simulink model "system_model"  (R2025b)
settings: Solver=VariableStepAuto  StartTime=0.0  StopTime=5  RelTol=1e-3
PreLoadFcn:
  | sideswipe_preload
  | sideswipe_config
InitFcn:
  | sideswipe_plant
values from neighbouring files (symbols this model uses):
  A1p = A1    [sideswipe_control.m]
  A2 = [0   1 ... (first row only)    [sideswipe_plant.m]
  a_v = Ts/(tau_v + Ts)    [sideswipe_control.m]
  accel_bias = 0    [sideswipe_control.m]
  accel_noise = 0    [sideswipe_control.m]
  alpha_comp = tau_cf/(tau_cf + Ts)    [sideswipe_control.m]
  B1p = [B1 Bd]    [sideswipe_control.m]
  B2 = [0    0 ... (first row only)    [sideswipe_plant.m]
  C1 = eye(4)    [sideswipe_plant.m]
  C2 = eye(2)    [sideswipe_plant.m]
  cotroller = 1    [sideswipe_control.m]
  D2 = zeros(2)    [sideswipe_plant.m]
  est_mode = 2    [sideswipe_control.m]
  g = 9.81    [sideswipe_params.m]
  gyro_bias = 0    [sideswipe_control.m]
  gyro_drift = 0    [sideswipe_control.m]
  gyro_noise = 0    [sideswipe_control.m]
  h = 0.130    (= 0.13)    [sideswipe_params.m]
  K_lqr = dlqr(s4d.A, s4d.B, QQ, RR)    [sideswipe_control.m]
  K_PWM = 42.5    [sideswipe_params.m]
  Kd_phi = 0.67    [sideswipe_control.m]
  Kd_psi_c = 8    [sideswipe_control.m]
  Kd_x = 0.02    [sideswipe_control.m]
  Ki_psi_c = 0    [sideswipe_control.m]
  Ki_x = 0.005    [sideswipe_control.m]
  Kp_phi = 21    [sideswipe_control.m]
  Kp_psi_c = 80    [sideswipe_control.m]
  Kp_x = 0.02    [sideswipe_control.m]
  n_delay = 0    [sideswipe_control.m]
  phi_dot_ref = 0    [sideswipe_control.m]
  Psi0 = deg2rad(5)    [sideswipe_params.m]
  psi_ref_max = deg2rad(10)    [sideswipe_control.m]
  R = 0.0325    [sideswipe_params.m]
  theta_dot_ref = 0    [sideswipe_control.m]
  Ts = 0.004    [sideswipe_params.m]
  V_dz = 0    [sideswipe_params.m]
  V_sat = 6    [sideswipe_control.m]
  W = 0.068    [sideswipe_params.m]
undefined symbols (not defined in the file or in its folder): DiscIntNeverNeededParam
libraries: simulink x7, simulink_extras x2, slpidlib x1
settings Model: Creator=shukv  LastModifiedBy=shukv

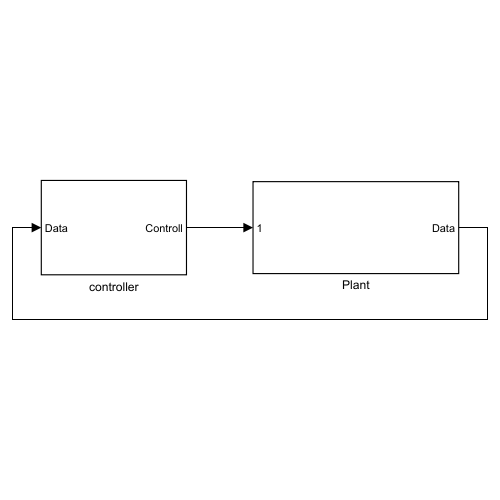
[thumbnail: Simulink's stored preview of the top-level diagram]
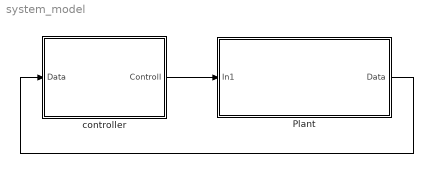
== system system_model ==
  Plant : Subsystem
  controller : Subsystem
  wires:
  controller/1(Controll) -> Plant/1(In1)
  Plant/1(Data) -> controller/1(Data)

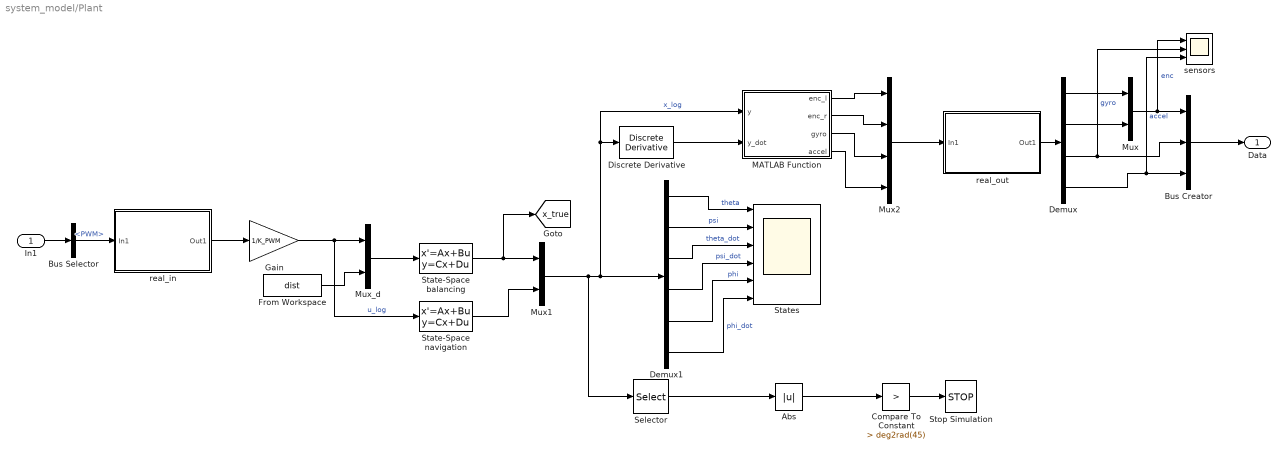
== system system_model/Plant ==
  In1 : Inport
  Abs : Abs  SaturateOnIntegerOverflow=off
  Bus Creator : BusCreator  Inputs=3  OutDataTypeStr=Bus: Data
  Bus Selector : BusSelector  OutputSignals=PWM
  Compare To Constant : simulink/Logic and Bit Operations/Compare To Constant  relop=>  const=deg2rad(45)  OutDataTypeStr=boolean
  Demux : Demux
  Demux1 : Demux  Outputs=6
  Discrete Derivative : simulink/Discrete/Discrete Derivative  gainval=1.0  ICPrevScaledInput=0.0  OutMin=[]  OutMax=[]  OutDataType=fixdt(1, 16)  OutScaling=2^-10  DoSatur=off
  From Workspace : FromWorkspace  VariableName=dist  SampleTime=Ts  Interpolate=off  OutputAfterFinalValue=Holding final value
  Gain : Gain  Gain=1/K_PWM
  MATLAB Function : MATLAB Function  TreatAsAtomicUnit=on
  Mux : Mux  Inputs=2
  Mux1 : Mux  Inputs=2
  Mux2 : Mux
  Mux_d : Mux  Inputs=2
  Selector : Selector  InputPortWidth=6  IndexOptions=Index vector (dialog)  Indices=2  OutputSizes=1
  State-Space balancing : StateSpace  A=A1p  B=B1p  C=C1  D=zeros(4,4)  InitialCondition=[0 Psi0 0 0]
  State-Space navigation : StateSpace  A=A2  B=B2  C=C2  D=D2  InitialCondition=0
  States : Scope  NumInputPorts=6
      settings: ActiveDisplayYMinimum=-1  ActiveDisplayYMaximum=1
  Stop Simulation : Stop
  real_in : Subsystem  Variant=on  EmptyChoice=on
  real_out : Subsystem  Variant=on  EmptyChoice=on
  sensors : Scope  NumInputPorts=3
      settings: ActiveDisplayYMinimum=-1  ActiveDisplayYMaximum=1
  Data : Outport
  tag scope: x_true=global
  wires:
  State-Space navigation/1 -> Mux1/2
  State-Space balancing/1 -> [x_true], Mux1/1
  In1/1 -> Bus Selector/1
  real_in/1(Out1) -> Gain/1
  Bus Selector/1 -> real_in/1(In1)  "<PWM>"
  MATLAB Function/1(enc_l) -> Mux2/1
  From Workspace/1 -> Mux_d/2
  Gain/1 -> State-Space navigation/1, Mux_d/1  "u_log"
  Mux_d/1 -> State-Space balancing/1
  Mux/1 -> sensors/1, Bus Creator/1  "enc"
  Mux1/1 -> Discrete Derivative/1, MATLAB Function/1(y), Demux1/1, Selector/1  "x_log"
  Discrete Derivative/1 -> MATLAB Function/2(y_dot)
  Demux/2 -> Mux/2
  Demux1/5 -> States/5  "phi"
  Demux1/1 -> States/1  "theta"
  Demux/3 -> sensors/2, Bus Creator/2  "gyro"
  Demux1/6 -> States/6  "phi_dot"
  Demux1/2 -> States/2  "psi"
  Demux1/3 -> States/3  "theta_dot"
  Demux1/4 -> States/4  "psi_dot"
  Selector/1 -> Abs/1
  MATLAB Function/2(enc_r) -> Mux2/2
  MATLAB Function/3(gyro) -> Mux2/3
  MATLAB Function/4(accel) -> Mux2/4
  Abs/1 -> Compare To Constant/1
  Mux2/1 -> real_out/1(In1)
  Bus Creator/1 -> Data/1
  Compare To Constant/1 -> Stop Simulation/1
  real_out/1(Out1) -> Demux/1
  Demux/1 -> Mux/1
  Demux/4 -> sensors/3, Bus Creator/3  "accel"

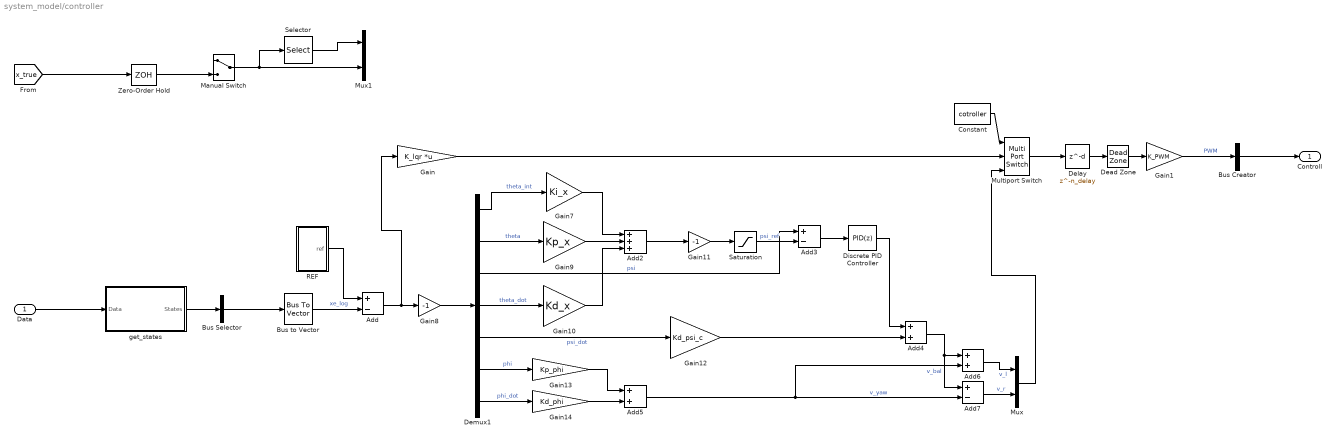
== system system_model/controller ==
  Data : Inport
  Add : Sum  Inputs=+-
  Add2 : Sum  Inputs=+++
  Add3 : Sum  Inputs=+-
  Add4 : Sum
  Add5 : Sum
  Add6 : Sum
  Add7 : Sum  Inputs=+-
  Bus Creator : BusCreator  Inputs=1  OutDataTypeStr=Bus: Controll
  Bus Selector : BusSelector  OutputSignals=theta_int,theta,psi,theta_dot,psi_dot,Phi,phi_dot  OutputAsBus=on
  Bus to Vector : BusToVector
  Constant : Constant  Value=cotroller
  Dead Zone : DeadZone  LowerValue=-V_dz  UpperValue=V_dz
  Delay : Delay  DelayLength=n_delay  SampleTime=Ts
  Demux1 : Demux  Outputs=7
  Discrete PID Controller : slpidlib/PID Controller  Controller=PID  Form=Parallel  TimeDomain=Discrete-time  UseExternalTs=off  SampleTime=Ts  IntegratorMethod=Forward Euler  FilterMethod=Forward Euler  ControllerParametersSource=internal  P=Kp_psi_c  I=Ki_psi_c  UseKiTs=off  D=0  UseExternalDerivativeSource=off  N=100  UseFilter=on  TunerSelectOption=Transfer Function Based (PID Tuner App)  InitialConditionSource=internal  InitialConditionForIntegrator=0  InitialConditionForFilter=0  DifferentiatorICPrevScaledInput=0  ExternalReset=none  TrackingMode=off  Kt=1  LimitOutput=off  SatLimitsSource=internal  UpperSaturationLimit=V_sat  LowerSaturationLimit=-V_sat  LinearizeAsGain=off  AntiWindupMode=clamping  Kb=1  LimitIntegrator=off  UpperIntegratorSaturationLimit=inf  LowerIntegratorSaturationLimit=-inf  POutMin=[]  POutMax=[]  IOutMin=[]  IOutMax=[]  DOutMin=[]  DOutMax=[]  NOutMin=[]  NOutMax=[]  SumOutMin=[]  SumOutMax=[]  SaturationOutMin=[]  SaturationOutMax=[]  PParamMin=[]  PParamMax=[]  IParamMin=[]  IParamMax=[]  DParamMin=[]  DParamMax=[]  NParamMin=[]  NParamMax=[]  KbParamMin=[]  KbParamMax=[]  KtParamMin=[]  KtParamMax=[]  KbOutMin=[]  KbOutMax=[]  KtOutMin=[]  KtOutMax=[]  IntegratorOutMin=[]  IntegratorOutMax=[]  FilterOutMin=[]  FilterOutMax=[]  SumI1OutMin=[]  SumI1OutMax=[]  SumI2OutMin=[]  SumI2OutMax=[]  SumI3OutMin=[]  SumI3OutMax=[]  SumI4OutMin=[]  SumI4OutMax=[]  SumDOutMin=[]  SumDOutMax=[]  DifferentiatorOutMin=[]  DifferentiatorOutMax=[]  FilterDiffOutCoefMin=[]  FilterDiffOutCoefMax=[]  ReciprocalOutMin=[]  ReciprocalOutMax=[]  SumDenOutMin=[]  SumDenOutMax=[]  SumNumOutMin=[]  SumNumOutMax=[]  DivideOutMin=[]  DivideOutMax=[]  UdiffTsProdOutMin=[]  UdiffTsProdOutMax=[]  NTsProdOutMin=[]  NTsProdOutMax=[]  UintegralTsProdOutMin=[]  UintegralTsProdOutMax=[]  UngainTsProdOutMin=[]  UngainTsProdOutMax=[]  ClampingZeroOutDataTypeStr=Inherit: Inherit via back propagation  ClampingZeroOutMin=[]  ClampingZeroOutMax=[]  FilterDenConstantOutDataTypeStr=Inherit: Inherit via back propagation  FilterDenConstantOutMin=[]  FilterDenConstantOutMax=[]  PCopyOutDataTypeStr=Inherit: Inherit via back propagation  PCopyOutMin=[]  PCopyOutMax=[]  NCopyOutDataTypeStr=Inherit: Inherit via back propagation  NCopyOutMin=[]  NCopyOutMax=[]  IntegratorContinuousStateAttributes=''  IntegratorStateMustResolveToSignalObject=off  IntegratorRTWStateStorageClass=Auto  FilterContinuousStateAttributes=''  FilterStateMustResolveToSignalObject=off  FilterRTWStateStorageClass=Auto  ParallelPVariant=InternalParameters  IdealPVariant=Disabled  IVariant=InternalParameters  DVariant=InternalParameters  IntegratorVariant=Discrete  SatVariant=Disabled  AWVariant=Passthrough  PCopyVariant=Disabled  TRVariant=Disabled  FdbkBlocksVariant=Forward  IdealPFdbkVariant=Disabled  SatFdbkVariant=Disabled  DerivativeFilterVariant=ForwardEulerFilter  NVariant=InternalParameters  NCopyVariant=Disabled  FilterICVariant=InternalICsFilter  IntegratorICVariant=InternalICs  ExternalResetVariant=Disabled  TRSumVariant=Passthrough  SumFdbkVariant=Disabled  SumVariant=Sum_PID  TsampFilterVariant=InternalTs  TsampNgainVariant=Passthrough  TsampIntegralVariant=Disabled_SignalSpec  ExternalSaturationOutDataTypeStr=Inherit: Same as second input  DerivativeSourceVariant=ErrorSignal  PreIntVariant=InternalPreInt
      settings: LibrarySourceBlock=simulink/Discrete/Discrete PID Controller
  Gain : Gain  Gain=K_lqr  Multiplication=Matrix(K*u)
  Gain1 : Gain  Gain=K_PWM
  Gain10 : Gain  Gain=Kd_x
  Gain11 : Gain  Gain=-1
  Gain12 : Gain  Gain=Kd_psi_c
  Gain13 : Gain  Gain=Kp_phi
  Gain14 : Gain  Gain=Kd_phi
  Gain7 : Gain  Gain=Ki_x
  Gain8 : Gain  Gain=-1
  Gain9 : Gain  Gain=Kp_x
  Manual Switch : ManualSwitch
  Multiport Switch : MultiPortSwitch  Inputs=2  SaturateOnIntegerOverflow=off  InputSameDT=off
  Mux : Mux  Inputs=2
  Mux1 : Mux  Inputs=2
  REF : Subsystem
  Saturation : Saturate  UpperLimit=psi_ref_max  LowerLimit=-psi_ref_max
  Selector : Selector  InputPortWidth=4  IndexOptions=Index vector (dialog)  Indices=1  OutputSizes=1
  Zero-Order Hold : ZeroOrderHold  SampleTime=Ts
  get_states : Subsystem
  Controll : Outport
  wires:
  Gain1/1 -> Bus Creator/1  "PWM"
  Add3/1 -> Discrete PID Controller/1
  Gain/1 -> Multiport Switch/2
  Bus Creator/1 -> Controll/1
  Add6/1 -> Mux/1  "v_l"
  [x_true] -> Zero-Order Hold/1
  Gain9/1 -> Add2/2
  Data/1 -> get_states/1(Data)
  Zero-Order Hold/1 -> Manual Switch/2
  Add5/1 -> Add7/2, Add6/2  "v_yaw"
  Add2/1 -> Gain11/1
  get_states/1(States) -> Bus Selector/1
  Manual Switch/1 -> Selector/1, Mux1/2
  Bus Selector/1 -> Bus to Vector/1
  Demux1/7 -> Gain14/1  "phi_dot"
  Selector/1 -> Mux1/1
  Discrete PID Controller/1 -> Add4/1
  Saturation/1 -> Add3/2  "psi_ref"
  Bus to Vector/1 -> Add/2  "xe_log"
  REF/1(ref) -> Add/1
  Gain13/1 -> Add5/1
  Demux1/6 -> Gain13/1  "phi"
  Add/1 -> Gain/1, Gain8/1
  Demux1/2 -> Gain9/1  "theta"
  Gain8/1 -> Demux1/1
  Demux1/1 -> Gain7/1  "theta_int"
  Demux1/3 -> Add3/1  "psi"
  Add4/1 -> Add6/1, Add7/1  "v_bal"
  Demux1/4 -> Gain10/1  "theta_dot"
  Demux1/5 -> Gain12/1  "psi_dot"
  Gain11/1 -> Saturation/1
  Gain7/1 -> Add2/1
  Gain10/1 -> Add2/3
  Gain14/1 -> Add5/2
  Gain12/1 -> Add4/2
  Add7/1 -> Mux/2  "v_r"
  Constant/1 -> Multiport Switch/1
  Mux/1 -> Multiport Switch/3
  Dead Zone/1 -> Gain1/1
  Multiport Switch/1 -> Delay/1
  Delay/1 -> Dead Zone/1

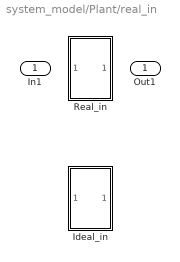
== system system_model/Plant/real_in ==
  In1 : Inport
  Ideal_in : Subsystem  VariantControl=(default)
  Real_in : Subsystem  VariantControl=real_model == 1
  Out1 : Outport

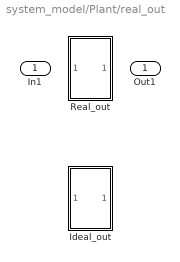
== system system_model/Plant/real_out ==
  In1 : Inport
  Ideal_out : Subsystem  VariantControl=(default)
  Real_out : Subsystem  VariantControl=real_model == 1
  Out1 : Outport

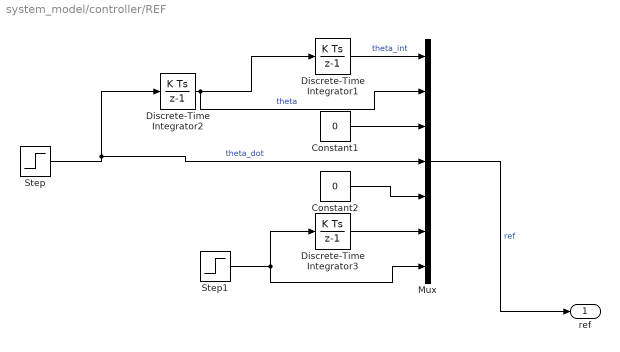
== system system_model/controller/REF ==
  Constant1 : Constant  Value=0
  Constant2 : Constant  Value=0
  Discrete-Time Integrator1 : DiscreteIntegrator  SampleTime=Ts  ICPrevOutput=DiscIntNeverNeededParam  ICPrevScaledInput=DiscIntNeverNeededParam
  Discrete-Time Integrator2 : DiscreteIntegrator  SampleTime=Ts  ICPrevOutput=DiscIntNeverNeededParam  ICPrevScaledInput=DiscIntNeverNeededParam
  Discrete-Time Integrator3 : DiscreteIntegrator  SampleTime=Ts  ICPrevOutput=DiscIntNeverNeededParam  ICPrevScaledInput=DiscIntNeverNeededParam
  Mux : Mux  Inputs=7
  Step : Step  After=theta_dot_ref  SampleTime=0
  Step1 : Step  After=phi_dot_ref  SampleTime=0
  ref : Outport
  wires:
  Mux/1 -> ref/1  "ref"
  Step1/1 -> Discrete-Time Integrator3/1, Mux/7
  Step/1 -> Mux/4, Discrete-Time Integrator2/1  "theta_dot"
  Constant1/1 -> Mux/3
  Discrete-Time Integrator2/1 -> Discrete-Time Integrator1/1, Mux/2  "theta"
  Discrete-Time Integrator1/1 -> Mux/1  "theta_int"
  Discrete-Time Integrator3/1 -> Mux/6
  Constant2/1 -> Mux/5

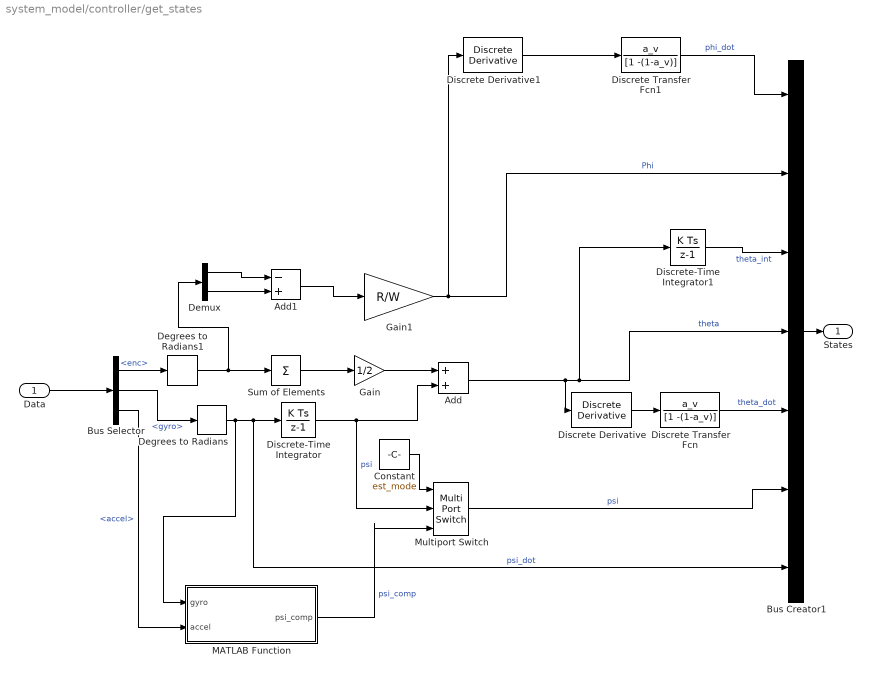
== system system_model/controller/get_states ==
  Data : Inport
  Add : Sum
  Add1 : Sum  Inputs=-+
  Bus Creator1 : BusCreator  Inputs=7
  Bus Selector : BusSelector  OutputSignals=enc,gyro,accel
  Constant : Constant  Value=est_mode
  Degrees to Radians : simulink_extras/Transformations/Degrees to Radians
  Degrees to Radians1 : simulink_extras/Transformations/Degrees to Radians
  Demux : Demux  Outputs=2
  Discrete Transfer Fcn : DiscreteTransferFcn  Numerator=a_v  Denominator=[1 -(1-a_v)]
  Discrete Transfer Fcn1 : DiscreteTransferFcn  Numerator=a_v  Denominator=[1 -(1-a_v)]
  Discrete Derivative : simulink/Discrete/Discrete Derivative  gainval=1.0  ICPrevScaledInput=0.0  OutMin=[]  OutMax=[]  OutDataType=fixdt(1, 16)  OutScaling=2^-10  DoSatur=off
  Discrete Derivative1 : simulink/Discrete/Discrete Derivative  gainval=1.0  ICPrevScaledInput=0.0  OutMin=[]  OutMax=[]  OutDataType=fixdt(1, 16)  OutScaling=2^-10  DoSatur=off
  Discrete-Time Integrator : DiscreteIntegrator  InitialCondition=Psi0  SampleTime=Ts  ICPrevOutput=DiscIntNeverNeededParam  ICPrevScaledInput=DiscIntNeverNeededParam
  Discrete-Time Integrator1 : DiscreteIntegrator  SampleTime=Ts  ICPrevOutput=DiscIntNeverNeededParam  ICPrevScaledInput=DiscIntNeverNeededParam
  Gain : Gain  Gain=1/2
  Gain1 : Gain  Gain=R/W
  MATLAB Function : MATLAB Function  TreatAsAtomicUnit=on
  Multiport Switch : MultiPortSwitch  Inputs=2  SaturateOnIntegerOverflow=off  InputSameDT=off
  Sum of Elements : Sum  Inputs=+
  States : Outport
  wires:
  Gain/1 -> Add/1
  Add/1 -> Discrete-Time Integrator1/1, Bus Creator1/4, Discrete Derivative/1  "theta"
  Degrees to Radians/1 -> MATLAB Function/1(gyro), Discrete-Time Integrator/1, Bus Creator1/7  "psi_dot"
  Sum of Elements/1 -> Gain/1
  Data/1 -> Bus Selector/1
  Bus Creator1/1 -> States/1
  Discrete-Time Integrator/1 -> Multiport Switch/2, Add/2  "psi"
  Degrees to Radians1/1 -> Demux/1, Sum of Elements/1
  Discrete Derivative/1 -> Discrete Transfer Fcn/1
  Bus Selector/2 -> Degrees to Radians/1  "<gyro>"
  Bus Selector/1 -> Degrees to Radians1/1  "<enc>"
  Discrete-Time Integrator1/1 -> Bus Creator1/3  "theta_int"
  Demux/1 -> Add1/1
  Demux/2 -> Add1/2
  Add1/1 -> Gain1/1
  Gain1/1 -> Bus Creator1/2, Discrete Derivative1/1  "Phi"
  Discrete Derivative1/1 -> Discrete Transfer Fcn1/1
  Bus Selector/3 -> MATLAB Function/2(accel)  "<accel>"
  MATLAB Function/1(psi_comp) -> Multiport Switch/3  "psi_comp"
  Constant/1 -> Multiport Switch/1
  Multiport Switch/1 -> Bus Creator1/6  "psi"
  Discrete Transfer Fcn/1 -> Bus Creator1/5  "theta_dot"
  Discrete Transfer Fcn1/1 -> Bus Creator1/1  "phi_dot"

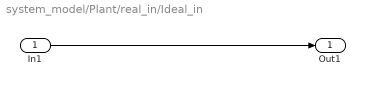
== system system_model/Plant/real_in/Ideal_in ==
  In1 : Inport
  Out1 : Outport
  wires:
  In1/1 -> Out1/1

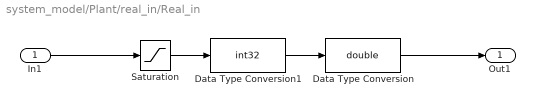
== system system_model/Plant/real_in/Real_in ==
  In1 : Inport
  Data Type Conversion : DataTypeConversion  OutDataTypeStr=double  SaturateOnIntegerOverflow=off  RndMeth=Floor
  Data Type Conversion1 : DataTypeConversion  OutDataTypeStr=int32  RndMeth=Nearest
  Saturation : Saturate  UpperLimit=V_sat*K_PWM  LowerLimit=-V_sat*K_PWM
  Out1 : Outport
  wires:
  Data Type Conversion1/1 -> Data Type Conversion/1
  Saturation/1 -> Data Type Conversion1/1
  Data Type Conversion/1 -> Out1/1
  In1/1 -> Saturation/1

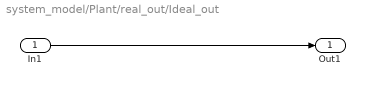
== system system_model/Plant/real_out/Ideal_out ==
  In1 : Inport
  Out1 : Outport
  wires:
  In1/1 -> Out1/1

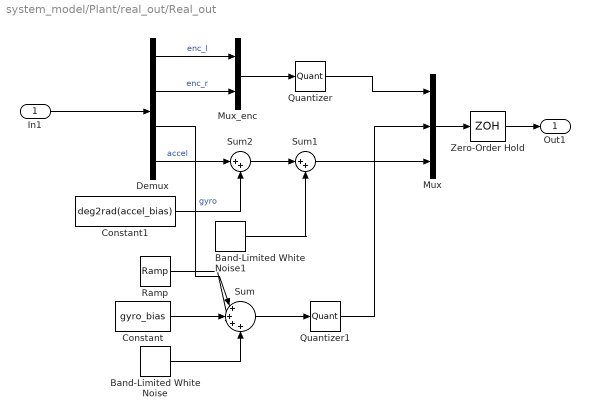
== system system_model/Plant/real_out/Real_out ==
  In1 : Inport
  Band-Limited White Noise : simulink/Sources/Band-Limited White Noise  Cov=gyro_noise^2*Ts  Ts=Ts  seed=[54321]
  Band-Limited White Noise1 : simulink/Sources/Band-Limited White Noise  Cov=(deg2rad(accel_noise))^2*Ts  Ts=Ts  seed=[23341]
  Constant : Constant  Value=gyro_bias
  Constant1 : Constant  Value=deg2rad(accel_bias)
  Demux : Demux
  Mux : Mux  Inputs=3
  Mux_enc : Mux  Inputs=2
  Quantizer : Quantizer  QuantizationInterval=enc_res
  Quantizer1 : Quantizer  QuantizationInterval=gyro_res
  Ramp : simulink/Sources/Ramp  slope=gyro_drift  start=0  InitialOutput=0
  Sum : Sum  Inputs=|++++
  Sum1 : Sum  Inputs=|++
  Sum2 : Sum  Inputs=|++
  Zero-Order Hold : ZeroOrderHold  SampleTime=Ts
  Out1 : Outport
  wires:
  In1/1 -> Demux/1
  Demux/1 -> Mux_enc/1  "enc_l"
  Ramp/1 -> Sum/3
  Demux/2 -> Mux_enc/2  "enc_r"
  Demux/3 -> Sum/1  "gyro"
  Demux/4 -> Sum2/1  "accel"
  Constant1/1 -> Sum2/2
  Constant/1 -> Sum/2
  Band-Limited White Noise/1 -> Sum/4
  Mux_enc/1 -> Quantizer/1
  Sum2/1 -> Sum1/1
  Band-Limited White Noise1/1 -> Sum1/2
  Sum/1 -> Quantizer1/1
  Quantizer/1 -> Mux/1
  Sum1/1 -> Mux/3
  Mux/1 -> Zero-Order Hold/1
  Zero-Order Hold/1 -> Out1/1
  Quantizer1/1 -> Mux/2

== matlab function system_model/controller/get_states/MATLAB Function ==
  settings: updateMethod=DISCRETE  sampleTime=Ts
  data: gyro input; psi_comp output; accel input; alpha_comp parameter; Ts parameter; Psi0 parameter
function psi_comp = comp_filter(gyro, accel, alpha_comp, Ts, Psi0)
   % Complementary filter: gyro for short-term, accelerometer for long-term
   persistent p
   if isempty(p)
       p = accel;                  % start at the initial tilt
   end
   p = alpha_comp*(p + gyro*Ts) + (1 - alpha_comp)*accel;
   psi_comp = p;

== matlab function system_model/Plant/MATLAB Function ==
  data: y input; y_dot input; enc_l output; enc_r output; gyro output; R parameter; W parameter; accel output; h parameter; g parameter
function [enc_l, enc_r, gyro, accel] = sensors(y,y_dot,R, W,h, g)
enc_l = rad2deg(y(1)- W/R/2 * y(5) -y(2));
enc_r = rad2deg(y(1)+ W/R/2 * y(5) -y(2));
gyro = rad2deg(y(4));
accel = y(2)- (R*y_dot(3)+h*y_dot(4))/g;
